simulink library "rotorcraft_lib"  (R2018b)
settings: Solver=VariableStepAuto  StartTime=0.0  StopTime=10.0  RelTol=1e-3
libraries: axes_transformation_lib x2, $bdroot x2, unit_conversions_lib x2
settings Model: Creator=root  LastModifiedBy=yannic
settings DataIOCC: ReturnWorkspaceOutputs=on

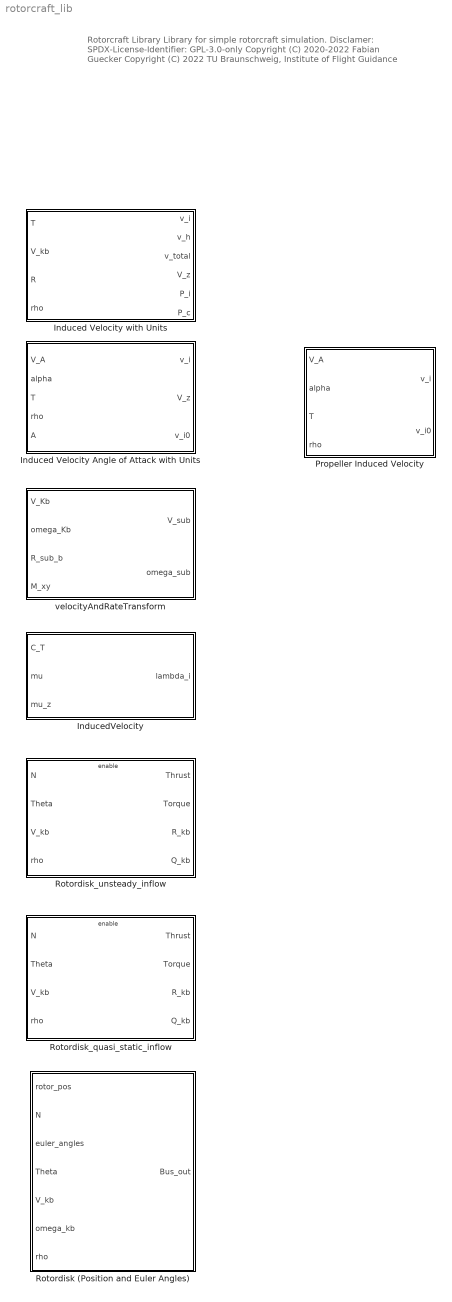
== system rotorcraft_lib ==
  note: Rotorcraft Library
      |
      | Library for simple rotorcraft simulation.
      |
      | Disclamer:
      | SPDX-License-Identifier: GPL-3.0-only
      |
      | Copyright (C) 2020-2022 Fabian Guecker
      | Copyright (C) 2022 TU Braunschweig, Institute of Flight Guidance
  Induced Velocity Angle of Attack with Units : MATLAB Function  TreatAsAtomicUnit=on
  Induced Velocity with Units : MATLAB Function  TreatAsAtomicUnit=on
  InducedVelocity : MATLAB Function  TreatAsAtomicUnit=on
  Propeller Induced Velocity : Subsystem  mask{F=0.0507}
      mask prompts: F "surface of the propeller, m-2"
      mask DialogControl DescGroupVar Prompt: Propeller Induced Velocity
      mask DialogControl DescTextVar Prompt: Computation of the induced velocity of the propeller
      mask DialogControl Control3 Prompt: Inputs:
      mask DialogControl Control4 Prompt: V_A    absolute velocity of the propeller relative to the air, m/s
      mask DialogControl Control5 Prompt: alpha    angle between the rotor plane and the velocity vector relative to the air, rad
      mask DialogControl Control6 Prompt: T    thrust, N
      mask DialogControl Control7 Prompt: rho    air density, kg/m-3
      mask DialogControl Control8 Prompt: F    surface of the propeller, m-2
      mask DialogControl Control10 Prompt: Outputs:
      mask DialogControl Control11 Prompt: v_i    induced velocity of the propeller, m/s
      mask DialogControl Control12 Prompt: v_i0    induced velocity for V_A = 0, m/s
  Rotordisk (Position and Euler Angles) : Subsystem  mask{R=0.9, chord=66.5 / 1000, Nb=2, C_l_alpha=5.75, C_d_0=0.0113, C_d_1=0, C_d_2=0.75, tau=0.01, lambda_i_inital=00, QS_Enable=on}
      mask prompts: R "Rotor Radius [m]"; chord "Blade Chord [m]"; Nb "Number of blades"; C_l_alpha "lift slope"; C_d_0 "Drag Coeff Cd_0"; C_d_1 "Drag Coeff Cd_1"; C_d_2 "Drag Coeff Cd_2"; tau "Inflow time constant [s]"; lambda_i_inital "Inital induced flow lambda_i"; QS_Enable "Quasi Static Inflow"
      mask TypeOptions R: OPT_Rotordisk/R
      mask TypeOptions chord: OPT_Rotordisk/chord
      mask TypeOptions Nb: OPT_Rotordisk/Nb
      mask TypeOptions C_l_alpha: OPT_Rotordisk/C_l_alpha
      mask TypeOptions C_d_0: OPT_Rotordisk/C_d_0
      mask TypeOptions C_d_1: OPT_Rotordisk/C_d_1
      mask TypeOptions C_d_2: OPT_Rotordisk/C_d_2
      mask TypeOptions tau: OPT_Rotordisk/tau
      mask TypeOptions lambda_i_inital: OPT_Rotordisk/inital_lambda_i
  Rotordisk_quasi_static_inflow : Subsystem  mask{R=0, chord=0, Nb=0, C_l_alpha=0, C_d_0=0, C_d_1=0, C_d_2=0, tau=0}
      mask prompts: R "Rotor Radius [m]"; chord "Blade Chord [m]"; Nb "Number of blades"; C_l_alpha "lift slope"; C_d_0 "Drag Coeff Cd_0"; C_d_1 "Drag Coeff Cd_1"; C_d_2 "Drag Coeff Cd_2"; tau "Inflow time constant [s]"
      mask init:
      | R>0;
      | chord>0;
      | Nb>0;
  Rotordisk_unsteady_inflow : Subsystem  mask{R=0.9, chord=0.0665, Nb=2, C_l_alpha=5.75, C_d_0=0, C_d_1=0, C_d_2=0, tau=0.3, inital_lambda_i=0}
      mask prompts: R "Rotor Radius [m]"; chord "Blade Chord [m]"; Nb "Number of blades"; C_l_alpha "lift slope"; C_d_0 "Drag Coeff Cd_0"; C_d_1 "Drag Coeff Cd_1"; C_d_2 "Drag Coeff Cd_2"; tau "Inflow time constant [s]"; inital_lambda_i "Inital induced flow lambda_i"
      mask init:
      | if(tau == 0)
      |     ssA = 0;
      |     ssB = 0;
      |     ssC = 0;
      |     ssD = 1;
      |     inital_value = inital_lambda_i; 
      | else
      |     ssA = -1/tau;
      |     ssB = 1;
      |     ssC = 1/tau;
      |     ssD = 0;
      |     inital_value = inital_lambda_i*tau;
      | end
  velocityAndRateTransform : MATLAB Function  TreatAsAtomicUnit=on

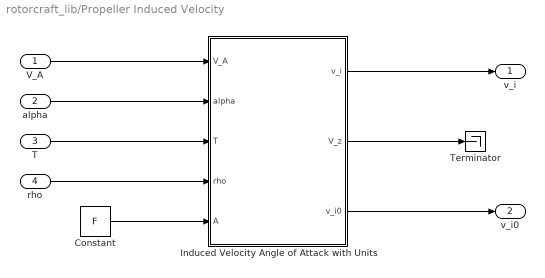
== system rotorcraft_lib/Propeller Induced Velocity ==
  V_A : Inport
  alpha : Inport  Port=2
  T : Inport  Port=3
  rho : Inport  Port=4
  Constant : Constant  Value=F
  Induced Velocity Angle of Attack with Units : MATLAB Function  TreatAsAtomicUnit=on
  Terminator : Terminator
  v_i : Outport
  v_i0 : Outport  Port=2
  wires:
  Constant/1 -> Induced Velocity Angle of Attack with Units/5(A)
  T/1 -> Induced Velocity Angle of Attack with Units/3(T)
  rho/1 -> Induced Velocity Angle of Attack with Units/4(rho)
  Induced Velocity Angle of Attack with Units/1(v_i) -> v_i/1
  Induced Velocity Angle of Attack with Units/2(V_z) -> Terminator/1
  Induced Velocity Angle of Attack with Units/3(v_i0) -> v_i0/1
  alpha/1 -> Induced Velocity Angle of Attack with Units/2(alpha)
  V_A/1 -> Induced Velocity Angle of Attack with Units/1(V_A)

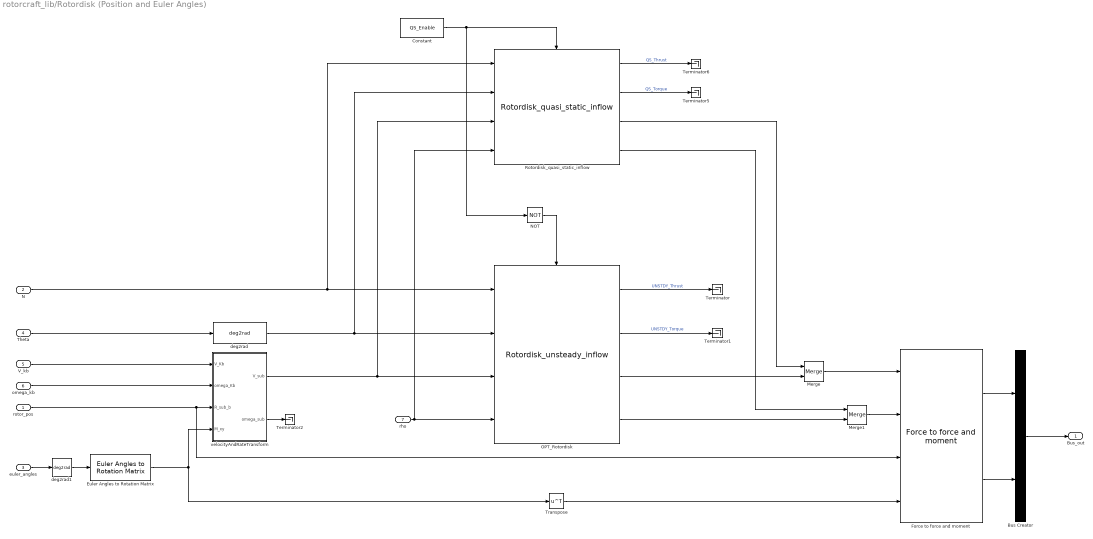
== system rotorcraft_lib/Rotordisk (Position and Euler Angles) ==
  rotor_pos : Inport
  N : Inport  Port=2
  euler_angles : Inport  Port=3
  Theta : Inport  Port=4
  V_kb : Inport  Port=5
  omega_kb : Inport  Port=6
  rho : Inport  Port=7
  Bus Creator : BusCreator  Inputs=2
  Constant : Constant  Value=QS_Enable
  Euler Angles to Rotation Matrix : axes_transformation_lib/Euler Angles to Rotation Matrix  SystemSampleTime=-1
      settings: SourceProductName=LADAC
  Force to force and moment : axes_transformation_lib/Force to force and moment  SystemSampleTime=-1
      settings: SourceProductName=LADAC
  Merge : Merge
  Merge1 : Merge
  NOT : Logic  Operator=NOT  IconShape=distinctive  AllPortsSameDT=off  OutDataTypeStr=boolean
  OPT_Rotordisk : $bdroot/Rotordisk_unsteady_inflow  R=R  chord=chord  Nb=Nb  C_l_alpha=C_l_alpha  C_d_0=C_d_0  C_d_1=C_d_1  C_d_2=C_d_2  tau=tau  inital_lambda_i=lambda_i_inital
  Rotordisk_quasi_static_inflow : $bdroot/Rotordisk_quasi_static_inflow  R=R  chord=chord  Nb=Nb  C_l_alpha=C_l_alpha  C_d_0=C_d_0  C_d_1=C_d_1  C_d_2=C_d_2  tau=tau
  Terminator{,1..2,5..6} (5 alike) : Terminator
  Transpose : Math  Operator=transpose  SaturateOnIntegerOverflow=on
  deg2rad : unit_conversions_lib/deg2rad
      settings: SourceProductName=LADAC
  deg2rad1 : unit_conversions_lib/deg2rad
      settings: SourceProductName=LADAC
  velocityAndRateTransform : MATLAB Function  TreatAsAtomicUnit=on
  Bus_out : Outport  VectorParamsAs1DForOutWhenUnconnected=on
  wires:
  euler_angles/1 -> deg2rad1/1
  Euler Angles to Rotation Matrix/1 -> velocityAndRateTransform/4(M_xy), Transpose/1
  V_kb/1 -> velocityAndRateTransform/1(V_Kb)
  Bus Creator/1 -> Bus_out/1
  Force to force and moment/2 -> Bus Creator/2
  Theta/1 -> deg2rad/1
  OPT_Rotordisk/2 -> Terminator1/1  "UNSTDY_Torque"
  rotor_pos/1 -> Force to force and moment/3, velocityAndRateTransform/3(R_sub_b)
  Force to force and moment/1 -> Bus Creator/1
  OPT_Rotordisk/1 -> Terminator/1  "UNSTDY_Thrust"
  omega_kb/1 -> velocityAndRateTransform/2(omega_Kb)
  Transpose/1 -> Force to force and moment/4
  velocityAndRateTransform/2(omega_sub) -> Terminator2/1
  deg2rad1/1 -> Euler Angles to Rotation Matrix/1
  N/1 -> Rotordisk_quasi_static_inflow/1, OPT_Rotordisk/1
  velocityAndRateTransform/1(V_sub) -> Rotordisk_quasi_static_inflow/3, OPT_Rotordisk/3
  rho/1 -> Rotordisk_quasi_static_inflow/4, OPT_Rotordisk/4
  deg2rad/1 -> Rotordisk_quasi_static_inflow/2, OPT_Rotordisk/2
  Constant/1 -> NOT/1, Rotordisk_quasi_static_inflow/Enable
  NOT/1 -> OPT_Rotordisk/Enable
  Rotordisk_quasi_static_inflow/1 -> Terminator6/1  "QS_Thrust"
  Rotordisk_quasi_static_inflow/2 -> Terminator5/1  "QS_Torque"
  Rotordisk_quasi_static_inflow/3 -> Merge/1
  Merge/1 -> Force to force and moment/1
  OPT_Rotordisk/3 -> Merge/2
  Merge1/1 -> Force to force and moment/2
  OPT_Rotordisk/4 -> Merge1/2
  Rotordisk_quasi_static_inflow/4 -> Merge1/1

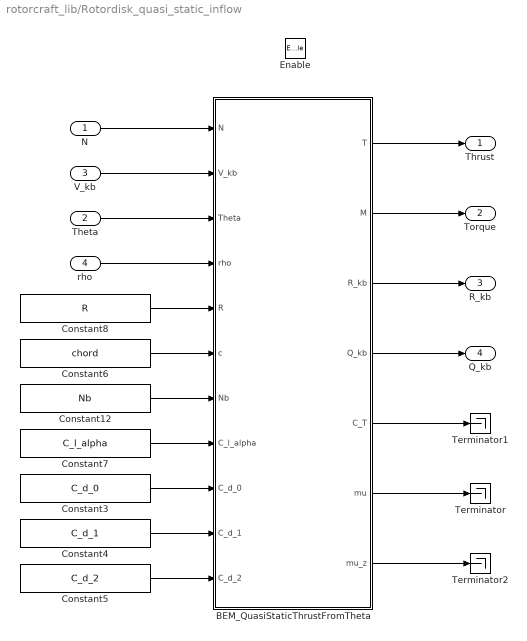
== system rotorcraft_lib/Rotordisk_quasi_static_inflow ==
  N : Inport
  Theta : Inport  Port=2
  V_kb : Inport  Port=3
  rho : Inport  Port=4
  Enable : EnablePort
  BEM_QuasiStaticThrustFromTheta : MATLAB Function  TreatAsAtomicUnit=on
  Constant12 : Constant  Value=Nb
  Constant3 : Constant  Value=C_d_0
  Constant4 : Constant  Value=C_d_1
  Constant5 : Constant  Value=C_d_2
  Constant6 : Constant  Value=chord
  Constant7 : Constant  Value=C_l_alpha
  Constant8 : Constant  Value=R
  Terminator : Terminator
  Terminator1 : Terminator
  Terminator2 : Terminator
  Thrust : Outport  VectorParamsAs1DForOutWhenUnconnected=on
  Torque : Outport  Port=2  VectorParamsAs1DForOutWhenUnconnected=on
  R_kb : Outport  Port=3  VectorParamsAs1DForOutWhenUnconnected=on
  Q_kb : Outport  Port=4  VectorParamsAs1DForOutWhenUnconnected=on
  wires:
  BEM_QuasiStaticThrustFromTheta/4(Q_kb) -> Q_kb/1
  BEM_QuasiStaticThrustFromTheta/3(R_kb) -> R_kb/1
  BEM_QuasiStaticThrustFromTheta/2(M) -> Torque/1
  BEM_QuasiStaticThrustFromTheta/1(T) -> Thrust/1
  rho/1 -> BEM_QuasiStaticThrustFromTheta/4(rho)
  V_kb/1 -> BEM_QuasiStaticThrustFromTheta/2(V_kb)
  Constant8/1 -> BEM_QuasiStaticThrustFromTheta/5(R)
  Constant6/1 -> BEM_QuasiStaticThrustFromTheta/6(c)
  Constant12/1 -> BEM_QuasiStaticThrustFromTheta/7(Nb)
  Constant5/1 -> BEM_QuasiStaticThrustFromTheta/11(C_d_2)
  Constant4/1 -> BEM_QuasiStaticThrustFromTheta/10(C_d_1)
  Constant3/1 -> BEM_QuasiStaticThrustFromTheta/9(C_d_0)
  Constant7/1 -> BEM_QuasiStaticThrustFromTheta/8(C_l_alpha)
  N/1 -> BEM_QuasiStaticThrustFromTheta/1(N)
  Theta/1 -> BEM_QuasiStaticThrustFromTheta/3(Theta)
  BEM_QuasiStaticThrustFromTheta/6(mu) -> Terminator/1
  BEM_QuasiStaticThrustFromTheta/5(C_T) -> Terminator1/1
  BEM_QuasiStaticThrustFromTheta/7(mu_z) -> Terminator2/1

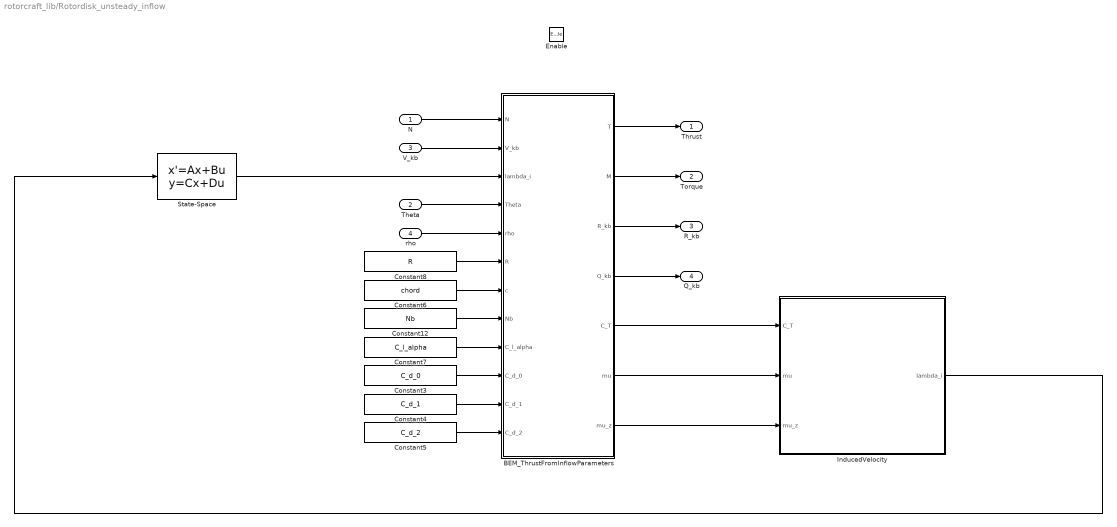
== system rotorcraft_lib/Rotordisk_unsteady_inflow ==
  N : Inport
  Theta : Inport  Port=2
  V_kb : Inport  Port=3
  rho : Inport  Port=4
  Enable : EnablePort
  BEM_ThrustFromInflowParameters : MATLAB Function  TreatAsAtomicUnit=on
  Constant12 : Constant  Value=Nb
  Constant3 : Constant  Value=C_d_0
  Constant4 : Constant  Value=C_d_1
  Constant5 : Constant  Value=C_d_2
  Constant6 : Constant  Value=chord
  Constant7 : Constant  Value=C_l_alpha
  Constant8 : Constant  Value=R
  InducedVelocity : MATLAB Function  TreatAsAtomicUnit=on
  State-Space : StateSpace  A=ssA  B=ssB  C=ssC  D=ssD  InitialCondition=inital_value
  Thrust : Outport  VectorParamsAs1DForOutWhenUnconnected=on
  Torque : Outport  Port=2  VectorParamsAs1DForOutWhenUnconnected=on
  R_kb : Outport  Port=3  VectorParamsAs1DForOutWhenUnconnected=on
  Q_kb : Outport  Port=4  VectorParamsAs1DForOutWhenUnconnected=on
  wires:
  Theta/1 -> BEM_ThrustFromInflowParameters/4(Theta)
  N/1 -> BEM_ThrustFromInflowParameters/1(N)
  BEM_ThrustFromInflowParameters/5(C_T) -> InducedVelocity/1(C_T)
  Constant7/1 -> BEM_ThrustFromInflowParameters/9(C_l_alpha)
  Constant3/1 -> BEM_ThrustFromInflowParameters/10(C_d_0)
  Constant4/1 -> BEM_ThrustFromInflowParameters/11(C_d_1)
  Constant5/1 -> BEM_ThrustFromInflowParameters/12(C_d_2)
  Constant12/1 -> BEM_ThrustFromInflowParameters/8(Nb)
  Constant6/1 -> BEM_ThrustFromInflowParameters/7(c)
  Constant8/1 -> BEM_ThrustFromInflowParameters/6(R)
  V_kb/1 -> BEM_ThrustFromInflowParameters/2(V_kb)
  rho/1 -> BEM_ThrustFromInflowParameters/5(rho)
  BEM_ThrustFromInflowParameters/1(T) -> Thrust/1
  BEM_ThrustFromInflowParameters/2(M) -> Torque/1
  BEM_ThrustFromInflowParameters/3(R_kb) -> R_kb/1
  BEM_ThrustFromInflowParameters/4(Q_kb) -> Q_kb/1
  BEM_ThrustFromInflowParameters/6(mu) -> InducedVelocity/2(mu)
  BEM_ThrustFromInflowParameters/7(mu_z) -> InducedVelocity/3(mu_z)
  InducedVelocity/1(lambda_i) -> State-Space/1
  State-Space/1 -> BEM_ThrustFromInflowParameters/3(lambda_i)

== matlab function rotorcraft_lib/InducedVelocity ==
  data: C_T input; lambda_i output; mu input; mu_z input
function lambda_i  = fcn(C_T, mu, mu_z)

[lambda_i] = inducedVelocity(C_T, mu, mu_z);

end

== matlab function rotorcraft_lib/Rotordisk_quasi_static_inflow/BEM_QuasiStaticThrustFromTheta ==
  data: N input; V_kb input; Theta input; rho input; R input; c input; Nb input; C_l_alpha input; T output; M output; R_kb output; Q_kb output; C_d_0 input; C_d_1 input; C_d_2 input; C_T output; mu output; mu_z output
function  [T, M, R_kb, Q_kb, C_T, mu, mu_z] = fcn(N, V_kb, Theta, rho, R, c, Nb, C_l_alpha, C_d_0, C_d_1, C_d_2)

[T, M, R_kb, Q_kb, C_T, mu, mu_z] = bemQuasiStaticThrustFromTheta(N, V_kb, Theta, rho, R, c, Nb, C_l_alpha, C_d_0, C_d_1, C_d_2);

end

== matlab function rotorcraft_lib/Rotordisk_unsteady_inflow/InducedVelocity ==
  data: C_T input; lambda_i output; mu input; mu_z input
function lambda_i  = fcn(C_T, mu, mu_z)

[lambda_i] = inducedVelocity(C_T, mu, mu_z);

end

== matlab function rotorcraft_lib/Rotordisk (Position and Euler Angles)/velocityAndRateTransform ==
  data: V_Kb input; V_sub output; omega_Kb input; R_sub_b input; M_xy input; omega_sub output
function [ V_sub, omega_sub ] = fcn(V_Kb, omega_Kb, R_sub_b, M_xy)

[ V_sub, omega_sub ] = velocityAndRateTransform(V_Kb, omega_Kb, R_sub_b, M_xy);

end

== matlab function rotorcraft_lib/Induced Velocity Angle of Attack with Units ==
  data: V_A input; v_i output; alpha input; T input; rho input; V_z output; A input; v_i0 output
function [ v_i, V_z, v_i0 ] = fcn( V_A, alpha, T, rho, A )

[ v_i, V_z, v_i0 ] = inducedVelocityWithUnitsAngleOfAttack( ...
    V_A, alpha, T, rho, A );

end

== matlab function rotorcraft_lib/Induced Velocity with Units ==
  data: T input; v_i output; V_kb input; R input; rho input; v_h output; v_total output; V_z output; P_i output; P_c output
function [v_i, v_h, v_total, V_z, P_i, P_c] = fcn(T, V_kb, R, rho)

[v_i, v_h, v_total, V_z, P_i, P_c] = ...
    inducedVelocityWithUnits(T, V_kb, R, rho);

end

== matlab function rotorcraft_lib/velocityAndRateTransform ==
  data: V_Kb input; V_sub output; omega_Kb input; R_sub_b input; M_xy input; omega_sub output
function [ V_sub, omega_sub ] = fcn(V_Kb, omega_Kb, R_sub_b, M_xy)

[ V_sub, omega_sub ] = velocityAndRateTransform(V_Kb, omega_Kb, R_sub_b, M_xy);

end

== matlab function rotorcraft_lib/Propeller Induced Velocity/Induced Velocity Angle of Attack with Units ==
  data: V_A input; v_i output; alpha input; T input; rho input; V_z output; A input; v_i0 output
function [ v_i, V_z, v_i0 ] = fcn( V_A, alpha, T, rho, A )

[ v_i, V_z, v_i0 ] = inducedVelocityWithUnitsAngleOfAttack( ...
    V_A, alpha, T, rho, A );

end

== matlab function rotorcraft_lib/Rotordisk_unsteady_inflow/BEM_ThrustFromInflowParameters ==
  data: N input; V_kb input; lambda_i input; Theta input; rho input; R input; c input; Nb input; C_l_alpha input; T output; M output; R_kb output; Q_kb output; C_d_0 input; C_d_1 input; C_d_2 input; C_T output; mu output; mu_z output
function  [T, M, R_kb, Q_kb, C_T, mu, mu_z] = fcn(N, V_kb, lambda_i, Theta, rho, R, c, Nb, C_l_alpha, C_d_0, C_d_1, C_d_2)

[T, M, R_kb, Q_kb, C_T, mu, mu_z] = bemThrustFromInflowParameters(N, V_kb, lambda_i, Theta, rho, R, c, Nb, C_l_alpha, C_d_0, C_d_1, C_d_2);

end
